simulink library "bat4s_lib"  (R2025b)
settings: Solver=VariableStepAuto  StartTime=0.0  StopTime=10.0  RelTol=1e-3
values from neighbouring files (symbols this model uses):
  bat4s = struct()    [bat4s_params.m]
undefined symbols (not defined in the file or in its folder): bat4s_params
libraries: fl_lib x19, nesl_utility x10, batt_lib x4
(part 1 of 2)
settings Model: Creator=SC-Br  LastModifiedBy=SC-Br

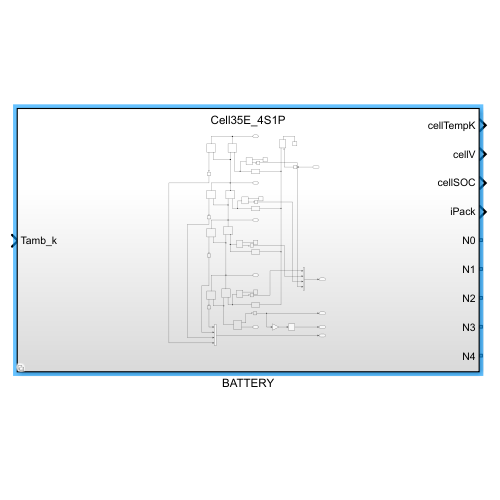
[thumbnail: Simulink's stored preview of the top-level diagram]
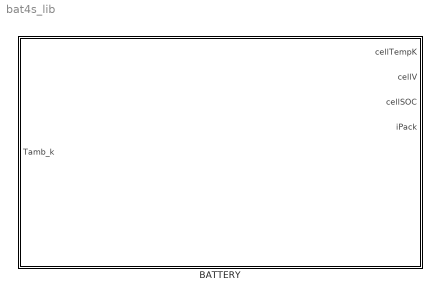
== system bat4s_lib ==
  BATTERY : Subsystem  Variant=on

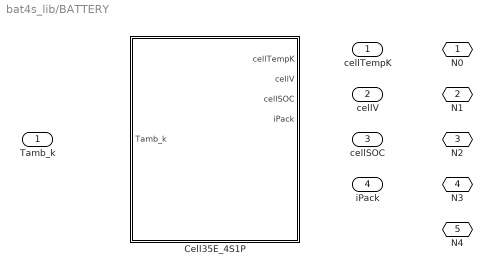
== system bat4s_lib/BATTERY ==
  Tamb_k : Inport
  Cell35E_4S1P : Subsystem  InitFcn=bat4s_params;  VariantControl=true
  N0 : PMIOPort  Side=Right
  N1 : PMIOPort  Port=2  Side=Right
  N2 : PMIOPort  Port=3  Side=Right
  N3 : PMIOPort  Port=4  Side=Right
  N4 : PMIOPort  Port=5  Side=Right
  cellTempK : Outport
  cellV : Outport  Port=2
  cellSOC : Outport  Port=3
  iPack : Outport  Port=4
